simulink model "furuta_urdf_test_LQR"  (R2025b)
settings: Solver=VariableStepAuto  StartTime=0.0  StopTime=10.0  RelTol=1e-3
settings Model: Creator=Compu  LastModifiedBy=theha

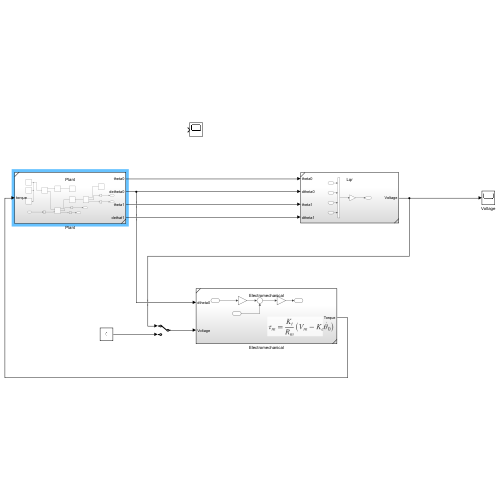
[thumbnail: Simulink's stored preview of the top-level diagram]
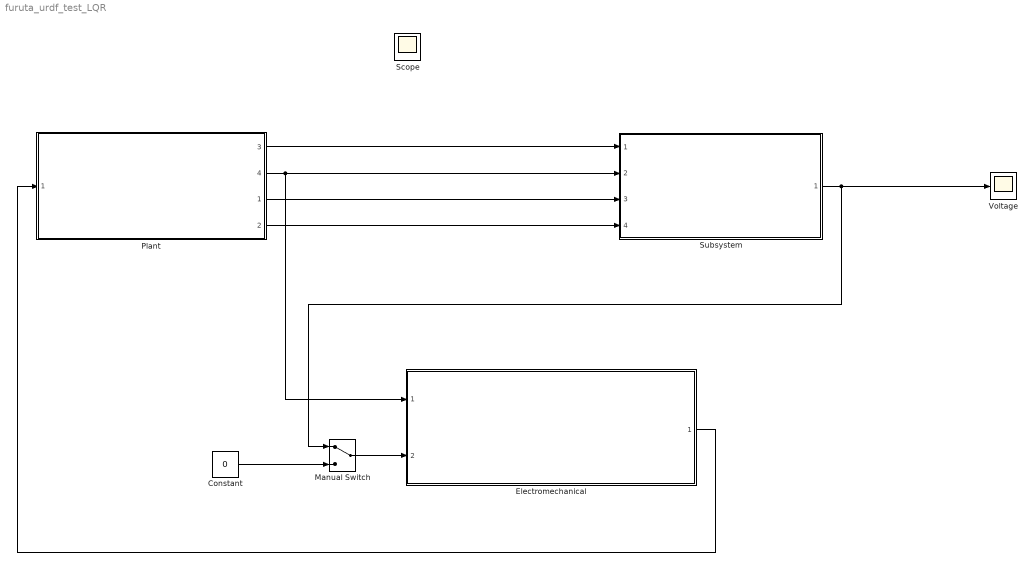
== system furuta_urdf_test_LQR ==
  Constant : Constant  Value=0
  Electromechanical : Subsystem  ReferencedSubsystem=Electromechanical
  Manual Switch : ManualSwitch
  Plant : Subsystem  ReferencedSubsystem=Plant
      settings: PortSchema="{\"entries\":[{\"content\":{\"sides\":[{\"content\":{\"connectorIds\":[\"In1\"]},\"type\":\"ConnectorPlacement.EquallySpacedRectSide\",\"uuid\":\"698e2142-6e18-4f9d-97c1-5a83dc679f38\"},{\"content\":{\"connectorIds\":[\"Out3\",\"Out4\",\"Out1\",\"Out2\"],\"side\":\"RIGHT\"},\"type\":\"ConnectorPlacement.EquallySpacedRectSide\",\"uuid\":\"8da0675e-fcb1-4bf9-9de6-c47ad67b018d\"},{\"content\":{\"side\":\"TOP\"},\"type\":\"ConnectorPlacement.EquallySpacedRectSide\",\"uuid\":\"bb61f6dc-b80a-4d58-a0df-5270abb20313\"}]},\"type\":\"ConnectorPlacement.EquallySpacedConnector\",\"uuid\":\"677f761d-6bde-4c02-9291-1daa9ae2b3af\"}],\"packageUris\":[\"http://schema.mathworks.com/mf0/Connector/R2020b\"],\"version\":\"1.0\"}"
  Scope : Scope
  Subsystem : Subsystem  ReferencedSubsystem=Lqr
  Voltage : Scope
      settings: ActiveDisplayYMinimum=-86.466235101222537  ActiveDisplayYMaximum=63.852491848707089  DataLoggingVariableName=ScopeData4
  wires:
  Plant/4 -> Subsystem/2, Electromechanical/1
  Electromechanical/1 -> Plant/1
  Plant/3 -> Subsystem/1
  Plant/1 -> Subsystem/3
  Plant/2 -> Subsystem/4
  Manual Switch/1 -> Electromechanical/2
  Constant/1 -> Manual Switch/2
  Subsystem/1 -> Voltage/1, Manual Switch/1
